simulink model "Grid_ModelSimVSGConB"  (R2025b)
settings: Solver=daessc  StartTime=0.0  StopTime=10  MaxStep=1e-5  RelTol=1e-3
InitFcn:
  | Grid_ModelSimV1
values from neighbouring files (symbols this model uses):
  a = 0.5    [Grid_ModelSimV1.m]
  b = (beta*gamma)/(beta + gamma - a)    [Grid_ModelSimV1.m]
  c = (beta + gamma - a)/mp    [Grid_ModelSimV1.m]
  D1 = Moh_Dp/Moh_Sbase    (= 0.2546)    [Grid_ModelSimV1.m]
  D2 = 0.4    [Grid_ModelSimV1.m]
  delta1_0 = delta1PCC0 + atan2(      P12_0*X1/V1PCCmag0,      V1PCCmag0 + Q12_0*X1/V1PCCmag0 )    [Grid_ModelSimV1.m]
  delta2_0 = delta2PCC0 + atan2(      Pm2_0*X2/V2PCCmag0,      V2PCCmag0 + Q21_0*X2/V2PCCmag0 )    [Grid_ModelSimV1.m]
  Dw1_0 = 0    [Grid_ModelSimV1.m]
  Dw2_0 = 0    [Grid_ModelSimV1.m]
  E2_0 = hypot(      Pm2_0*X2/V2PCCmag0,      V2PCCmag0 + Q21_0*X2/V2PCCmag0 )    [Grid_ModelSimV1.m]
  H1 = J*omega_nom^2/2    (= 39.9916370332)    [Grid_ModelSimV1.m]
  H2 = 12    [Grid_ModelSimV1.m]
  Imax = 1.20    (= 1.2)    [Grid_ModelSimV1.m]
  J = Moh_J/Moh_Sbase    (= 0.0008104)    [Grid_ModelSimV1.m]
  Ki = 0.5    [Grid_ModelSimV1.m]
  Kiq = Moh_Kiq*Moh_Sbase/Moh_Vbase    [Grid_ModelSimV1.m]
  Lf = 1e-3    (= 0.001)    [Grid_ModelSimV1.m]
  LimitEnable = 1    [Grid_ModelSimV1.m]
  Ls = Xs/ws    [Grid_ModelSimV1.m]
  Ls_line = Xs_line/ws    [Grid_ModelSimV1.m]
  nq = Moh_nq*Moh_Sbase/Moh_Vbase    [Grid_ModelSimV1.m]
  omega_nom = ws    (= 314.159265359)    [Grid_ModelSimV1.m]
  Pload_0 = P12_0    (= 1)    [Grid_ModelSimV1.m]
  Qref = 0.0    (= 0)    [Grid_ModelSimV1.m]
  Rf = 1.0    (= 1)    [Grid_ModelSimV1.m]
  RLFault = 0    [Grid_ModelSimV1.m]
  Rs = Zs_mag/sqrt(1 + XR_grid^2)    [Grid_ModelSimV1.m]
  Rs_line = GridLineFraction*Rs    [Grid_ModelSimV1.m]
  SolidFault = 0    [Grid_ModelSimV1.m]
  ws = 2*pi*f    (= 314.159265359)    [Grid_ModelSimV1.m]
  X1 = Xtf_src_total_pu    (= 0.15)    [Grid_ModelSimV1.m]
libraries: nesl_utility x87, ee_lib x78, fl_lib x40, eePowerMeasurement x7
(part 3 of 6)

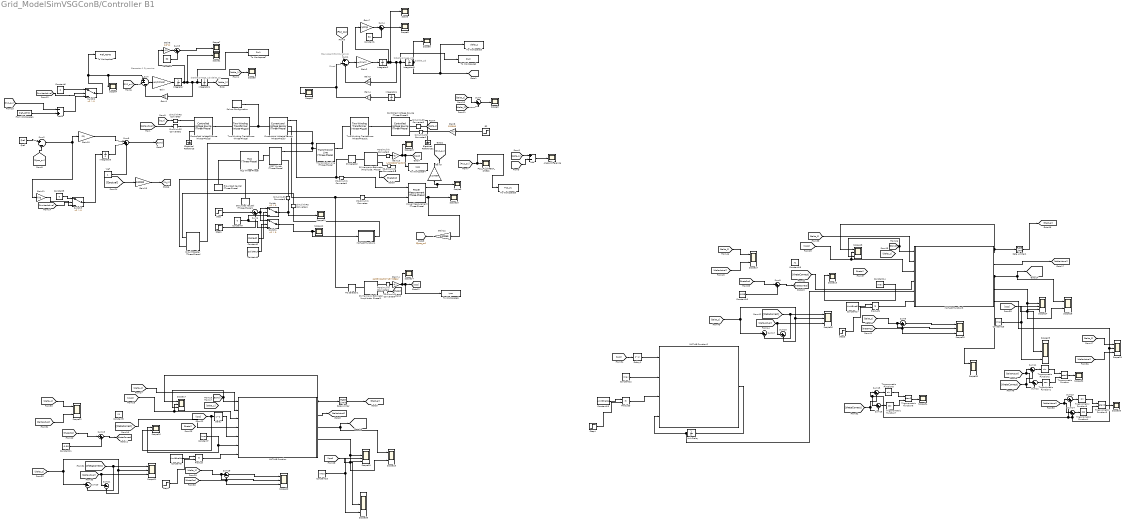
== system Grid_ModelSimVSGConB/Controller B1 ==
  note: Pload
  note: Equivalent Grid Dynamics
  note: $\delta_1$
  note: $\Delta\omega_1$
  note: Generator 1 Dynamics
  note: $\Delta\omega_2$
  note: $\delta_2$
  Add : Sum  Inputs=+-
  Add3 : Sum  Inputs=-+
  Angle Difference : Scope
      settings: ActiveDisplayYMinimum=-1797.079300536021  ActiveDisplayYMaximum=1392.8706624711849  DataLoggingVariableName=ScopeData11
  Circuit Breaker (Three-Phase) : ee_lib/Switches & Breakers/Circuit Breaker (Three-Phase)  R_closed=0.001 Ohm  G_open=1e-6 1/Ohm  threshold=0.5 V  breaker_behavior=ee.enum.switches.breakerBehavior.zeroCrossingEnable
      settings: InternalSimscapePortConfiguration="{\"Bottom\":[],\"Left\":[{\"id\":\"vT\",\"label\":\"vT\",\"type\":\"input\"},{\"id\":\"N1\",\"label\":\"~1\",\"type\":\"foundation.electrical.three_phase\"}],\"Right\":[{\"id\":\"N2\",\"label\":\"~2\",\"type\":\"foundation.electrical.three_phase\"}],\"Top\":[]}"
  Constant : Constant  Value=50
  Constant1 : Constant  Value=50
  Constant{7,10,12,14..15} (5 alike) : Constant  Value=Imax
  Constant11 : Constant  Value=-0.58
  Constant13 : Constant  Value=LimitEnable
  Constant16 : Constant  Value=-0.58
  Constant17 : Constant  Value=LimitEnable
  Constant18 : Constant  Value=X1
  Constant2 : Constant  Value=RLFault
  Constant3 : Constant  Value=SolidFault
  Constant4 : Constant  Value=0
  Constant5 : Constant  Value=0
  Constant6 : Constant  Value=0
  Constant8 : Constant  Value=LimitEnable
  Constant9 : Constant  Value=X1
  Controlled Voltage Source (Three-Phase) : ee_lib/Sources/Controlled Voltage Source (Three-Phase)  input_option=ee.enum.inputType.singleFreqAC  FRated=50 Hz
      settings: InternalSimscapePortConfiguration="{\"Bottom\":[],\"Left\":[{\"id\":\"Vt\",\"label\":\"Vt\",\"type\":\"input\"},{\"id\":\"ph\",\"label\":\"ph\",\"type\":\"input\"},{\"id\":\"n\",\"label\":\"n\",\"type\":\"foundation.electrical.electrical\"}],\"Right\":[{\"id\":\"N\",\"label\":\"~\",\"type\":\"foundation.electrical.three_phase\"}],\"Top\":[]}"
  Controlled Voltage Source (Three-Phase)1 : ee_lib/Sources/Controlled Voltage Source (Three-Phase)  input_option=ee.enum.inputType.singleFreqAC  FRated=50 Hz
      settings: InternalSimscapePortConfiguration="{\"Bottom\":[],\"Left\":[{\"id\":\"Vt\",\"label\":\"Vt\",\"type\":\"input\"},{\"id\":\"ph\",\"label\":\"ph\",\"type\":\"input\"},{\"id\":\"n\",\"label\":\"n\",\"type\":\"foundation.electrical.electrical\"}],\"Right\":[{\"id\":\"N\",\"label\":\"~\",\"type\":\"foundation.electrical.three_phase\"}],\"Top\":[]}"
  Current and Voltage Sensor (Three-Phase) : ee_lib/Sensors & Transducers/Current and Voltage Sensor (Three-Phase)  vMeasurementType=ee.enum.vmeasurement.ll  outputUnit=ee.enum.unit.si  SRated=100e6 A*V  VRated=24e3 V  I_specify=off  I_priority=None  I=[0, 0, 0] A  I_nominal_specify=off  I_nominal_value=1  I_nominal_unit=A  V_specify=off  V_priority=None  V=[0, 0, 0] V  V_nominal_specify=off  V_nominal_value=1  V_nominal_unit=V
      settings: InternalSimscapePortConfiguration="{\"Bottom\":[],\"Left\":[{\"id\":\"N1\",\"label\":\"~1\",\"type\":\"foundation.electrical.three_phase\"}],\"Right\":[{\"id\":\"V_output\",\"label\":\"V\",\"type\":\"output\"},{\"id\":\"I_output\",\"label\":\"I\",\"type\":\"output\"},{\"id\":\"N2\",\"label\":\"~2\",\"type\":\"foundation.electrical.three_phase\"}],\"Top\":[]}"
  Delay : Delay  InitialCondition=1  SampleTime=1e-4
  Delay1 : Delay  InitialCondition=1  SampleTime=1e-4
  E2 : Step  Before=E2_0  After=E2_0  SampleTime=0
  Electrical Reference : fl_lib/Electrical/Electrical Elements/Electrical Reference
  Electrical Reference1 : fl_lib/Electrical/Electrical Elements/Electrical Reference
  From Workspace1 : FromWorkspace  VariableName=Pref_AEMO  Interpolate=off  OutputAfterFinalValue=Holding final value
  Gain : Gain  Gain=ws/(2*H1)
  Gain1 : Gain  Gain=D1
  Gain10 : Gain  Gain=nq
  Gain11 : Gain  Gain=Kiq
  Gain12 : Gain  Gain=1/100e6
  Gain13 : Gain  Gain=1/(132000*sqrt(2))
  Gain14 : Gain  Gain=sqrt(3)/(sqrt(2)*437.3866)
  Gain15 : Gain  Gain=132000
  Gain2 : Gain  Gain=ws/(2*H2)
  Gain3 : Gain  Gain=D2
  Gain4 : Gain  Gain=Ki
  Gain5 : Gain  Gain=1/100e6
  Gain6 : Gain  Gain=1/2*pi
  Gain7 : Gain  Gain=1/2*pi
  Gain8 : Gain  Gain=132000
  Grounded Neutral (Three-Phase) : ee_lib/Connectors & References/Grounded Neutral (Three-Phase)
  Grounded Neutral (Three-Phase)1 : ee_lib/Connectors & References/Grounded Neutral (Three-Phase)
  Integrator : Integrator  InitialCondition=Dw1_0
  Integrator1 : Integrator  InitialCondition=delta1_0
  Integrator2 : Integrator  InitialCondition=Dw2_0
  Integrator3 : Integrator  InitialCondition=delta2_0
  Integrator4 : Integrator  InitialCondition=Pload_0/Ki
  Integrator5 : Integrator
  MATLAB Function : MATLAB Function  TreatAsAtomicUnit=on
  MATLAB Function1 : MATLAB Function  TreatAsAtomicUnit=on
  MATLAB Function2 : MATLAB Function  TreatAsAtomicUnit=on
  MATLAB Function3 : MATLAB Function  TreatAsAtomicUnit=on
  P12_PU_DIRECT_CHECK : Scope
      settings: ActiveDisplayYMinimum=0.025769954116994787  ActiveDisplayYMaximum=1.1382760295145928  DataLoggingVariableName=ScopeData3
  "PS Harmonic Estimator (Amplitude, Phase)" : fl_lib/Physical Signals/Periodic Operators/PS Harmonic Estimator (Amplitude, Phase)  f0=50 Hz  n=1  amplMin=0.001 V
      settings: InternalSimscapePortConfiguration="{\"Bottom\":[],\"Left\":[{\"id\":\"I\",\"label\":\"I\",\"type\":\"input\"}],\"Right\":[{\"id\":\"A\",\"label\":\"A\",\"type\":\"output\"},{\"id\":\"Phi\",\"label\":\"Phi\",\"type\":\"output\"}],\"Top\":[]}"
  "PS Harmonic Estimator (Amplitude, Phase)1" : fl_lib/Physical Signals/Periodic Operators/PS Harmonic Estimator (Amplitude, Phase)  f0=50 Hz  n=1  amplMin=0.001 A
      settings: InternalSimscapePortConfiguration="{\"Bottom\":[],\"Left\":[{\"id\":\"I\",\"label\":\"I\",\"type\":\"input\"}],\"Right\":[{\"id\":\"A\",\"label\":\"A\",\"type\":\"output\"},{\"id\":\"Phi\",\"label\":\"Phi\",\"type\":\"output\"}],\"Top\":[]}"
  PS Selector : fl_lib/Physical Signals/Nonlinear Operators/PS Selector  ix=1
      settings: InternalSimscapePortConfiguration="{\"Bottom\":[],\"Left\":[{\"id\":\"I\",\"label\":\"\",\"type\":\"input\"}],\"Right\":[{\"id\":\"O\",\"label\":\"\",\"type\":\"output\"}],\"Top\":[]}"
  PS Selector1 : fl_lib/Physical Signals/Nonlinear Operators/PS Selector  ix=1
      settings: InternalSimscapePortConfiguration="{\"Bottom\":[],\"Left\":[{\"id\":\"I\",\"label\":\"\",\"type\":\"input\"}],\"Right\":[{\"id\":\"O\",\"label\":\"\",\"type\":\"output\"}],\"Top\":[]}"
  PS-Simulink Converter{,1..5} (6 alike) : nesl_utility/PS-Simulink Converter  PhysicalDomain=network_engine_domain  SubClassName=ps_output  LeftPortType=input  RightPortType=output  PseudoPeriodic=off  Frequencies=[]  VectorFormat=inherit  Unit=inherit  AffineConversion=off
  Power Measurement (Three-Phase) : eePowerMeasurement/Power Measurement (Three-Phase)  LabelModeActiveChoice=Continuous  F=50  K=1  Seq=Positive  Ts=0
  Product : Product
  Product1 : Product
  Product3 : Product
  Qref : Constant  Value=Qref
  RLC (Three-Phase) : ee_lib/Passive/RLC Assemblies/RLC (Three-Phase)  port_option=ee.enum.threePhasePort.composite  component_structure=ee.enum.rlc.structure.SeriesRL  R=Rf Ohm  L=Lf H  C=1e-6 F  R_parasitic=0 Ohm  G_parasitic=0 1/Ohm  IL_specify=off  IL_priority=High  IL=[0, 0, 0] A  IL_nominal_specify=off  IL_nominal_value=1  IL_nominal_unit=A  VC_specify=off  VC_priority=High  VC=[0, 0, 0] V  VC_nominal_specify=off  VC_nominal_value=1  VC_nominal_unit=V
      settings: InternalSimscapePortConfiguration="{\"Bottom\":[],\"Left\":[{\"id\":\"N1\",\"label\":\"~1\",\"type\":\"foundation.electrical.three_phase\"}],\"Right\":[{\"id\":\"N2\",\"label\":\"~2\",\"type\":\"foundation.electrical.three_phase\"}],\"Top\":[]}"
  Rate Limiter : RateLimiter  RisingSlewLimit=5  FallingSlewLimit=-1000  SampleTimeMode=inherited
  Rate Limiter1 : RateLimiter  RisingSlewLimit=5  FallingSlewLimit=-1000  SampleTimeMode=inherited
  SPST Switch (Three-Phase) : ee_lib/Switches & Breakers/SPST Switch (Three-Phase)  R_closed=0.001 Ohm  G_open=1e-6 1/Ohm  threshold=0.5 V  i_vT_specify=off  i_vT_priority=None  i_vT=0 A  i_vT_nominal_specify=off  i_vT_nominal_value=1  i_vT_nominal_unit=A  I_specify=off  I_priority=None  I=[0, 0, 0] A  I_nominal_specify=off  I_nominal_value=1  I_nominal_unit=A  V_specify=off  V_priority=None  V=[0, 0, 0] V  V_nominal_specify=off  V_nominal_value=1  V_nominal_unit=V  i_a_specify=off  i_a_priority=None  i_a=0 A  i_a_nominal_specify=off  i_a_nominal_value=1  i_a_nominal_unit=A  v_a_specify=off  v_a_priority=None  v_a=0 V  v_a_nominal_specify=off  v_a_nominal_value=1  v_a_nominal_unit=V  i_b_specify=off  i_b_priority=None  i_b=0 A  i_b_nominal_specify=off  i_b_nominal_value=1  i_b_nominal_unit=A  v_b_specify=off  v_b_priority=None  v_b=0 V  v_b_nominal_specify=off  v_b_nominal_value=1  v_b_nominal_unit=V  i_c_specify=off  i_c_priority=None  i_c=0 A  i_c_nominal_specify=off  i_c_nominal_value=1  i_c_nominal_unit=A  v_c_specify=off  v_c_priority=None  v_c=0 V  v_c_nominal_specify=off  v_c_nominal_value=1  v_c_nominal_unit=V
      settings: InternalSimscapePortConfiguration="{\"Bottom\":[],\"Left\":[{\"id\":\"vT\",\"label\":\"vT\",\"type\":\"input\"},{\"id\":\"N1\",\"label\":\"~1\",\"type\":\"foundation.electrical.three_phase\"}],\"Right\":[{\"id\":\"N2\",\"label\":\"~2\",\"type\":\"foundation.electrical.three_phase\"}],\"Top\":[]}"
  Scope{,1..14,32..34} (18 alike) : Scope
      Scope10 settings: ActiveDisplayYMinimum=-7.0875379074731711E+6  ActiveDisplayYMaximum=3.5866343126415364E+7  DataLoggingVariableName=ScopeData10
      Scope11 settings: ActiveDisplayYMinimum=-1  ActiveDisplayYMaximum=1  DataLoggingVariableName=ScopeData12
      Scope12 settings: ActiveDisplayYMinimum=-0.099895670318205565  ActiveDisplayYMaximum=1.090580520157985  DataLoggingVariableName=ScopeData13
      Scope13 settings: ActiveDisplayYMinimum=-2.5658886223026931  ActiveDisplayYMaximum=3.94553749363296  DataLoggingVariableName=ScopeData17
      Scope14 settings: ActiveDisplayYMinimum=-1.0313612715858387  ActiveDisplayYMaximum=9.28225144427255  DataLoggingVariableName=ScopeData49
      Scope2 settings: ActiveDisplayYMinimum=-1.1623447136135812  ActiveDisplayYMaximum=1.3781315704633705  DataLoggingVariableName=ScopeData2
      Scope3 settings: ActiveDisplayYMinimum=-6.9165953549105517  ActiveDisplayYMaximum=7.2970312476918844  DataLoggingVariableName=ScopeData23
      Scope32 settings: ActiveDisplayYMinimum=-3.9269892876580919  ActiveDisplayYMaximum=3.9269891159141448  DataLoggingVariableName=ScopeData60
      Scope33 settings: ActiveDisplayYMinimum=-1  ActiveDisplayYMaximum=1  DataLoggingVariableName=ScopeData61
      Scope34 settings: ActiveDisplayYMinimum=-1.4401977699145856  ActiveDisplayYMaximum=2.6200072427590877  DataLoggingVariableName=ScopeData62
      Scope4 settings: ActiveDisplayYMinimum=-0.10712539123630682  ActiveDisplayYMaximum=1.1397496087636934  DataLoggingVariableName=ScopeData4
      Scope5 settings: ActiveDisplayYMinimum=-0.5315157226665419  ActiveDisplayYMaximum=2.1795261958257051  DataLoggingVariableName=ScopeData5
      Scope6 settings: DataLoggingVariableName=ScopeData6
      Scope7 settings: ActiveDisplayYMinimum=49.687624753361064  ActiveDisplayYMaximum=50.693198364995283  DataLoggingVariableName=ScopeData7
      Scope8 settings: ActiveDisplayYMinimum=49.92788610274394  ActiveDisplayYMaximum=50.170097472488152  DataLoggingVariableName=ScopeData8
      Scope9 settings: ActiveDisplayYMinimum=-1.0746752531857479E+8  ActiveDisplayYMaximum=3.4916793473002666E+8  DataLoggingVariableName=ScopeData9
  Scope{15..16,22..23,27..28,30} (7 alike) : Scope  NumInputPorts=2
      Scope15 settings: ActiveDisplayYMinimum=-1.1863011737345548  ActiveDisplayYMaximum=10.676710563610996  DataLoggingVariableName=ScopeData50
      Scope16 settings: ActiveDisplayYMinimum=-1.1863011737345548  ActiveDisplayYMaximum=10.676710563610996  DataLoggingVariableName=ScopeData63
      Scope22 settings: ActiveDisplayYMinimum=-0.789059573220128  ActiveDisplayYMaximum=0.68498191992001933  DataLoggingVariableName=ScopeData68
      Scope23 settings: ActiveDisplayYMinimum=-0.12499999999999997  ActiveDisplayYMaximum=1.125  DataLoggingVariableName=ScopeData69
      Scope27 settings: ActiveDisplayYMinimum=-3.7225747393161841  ActiveDisplayYMaximum=4.13168438536474  DataLoggingVariableName=ScopeData55
      Scope28 settings: ActiveDisplayYMinimum=-0.12499999999999997  ActiveDisplayYMaximum=1.125  DataLoggingVariableName=ScopeData56
      Scope30 settings: ActiveDisplayYMinimum=-0.12499999999999997  ActiveDisplayYMaximum=1.125  DataLoggingVariableName=ScopeData58
  Scope{17..18,20..21,25..26,29,31,35} (9 alike) : Scope  NumInputPorts=3
      Scope17 settings: ActiveDisplayYMinimum=-0.15152887647529475  ActiveDisplayYMaximum=1.3637598882776532  DataLoggingVariableName=ScopeData64
      Scope18 settings: ActiveDisplayYMinimum=-0.12862546618818504  ActiveDisplayYMaximum=1.1576291956936657  DataLoggingVariableName=ScopeData51
      Scope20 settings: ActiveDisplayYMinimum=-2.6035343832796971  ActiveDisplayYMaximum=9.8526279409331341  DataLoggingVariableName=ScopeData66
      Scope21 settings: ActiveDisplayYMinimum=-2.7720251649113785  ActiveDisplayYMaximum=1.647845241487004  DataLoggingVariableName=ScopeData67
      Scope25 settings: ActiveDisplayYMinimum=-2.6035343832796971  ActiveDisplayYMaximum=9.8526279409331341  DataLoggingVariableName=ScopeData53
      Scope26 settings: ActiveDisplayYMinimum=-2.7720251649113785  ActiveDisplayYMaximum=1.647845241487004  DataLoggingVariableName=ScopeData54
      Scope29 settings: ActiveDisplayYMinimum=-0.5707391589619073  ActiveDisplayYMaximum=5.1366524306571666  DataLoggingVariableName=ScopeData57
      Scope31 settings: ActiveDisplayYMinimum=-2.7504004579249388  ActiveDisplayYMaximum=0.52931298913436242  DataLoggingVariableName=ScopeData59
      Scope35 settings: ActiveDisplayYMinimum=-1.0836921534712509  ActiveDisplayYMaximum=9.974041191278685  DataLoggingVariableName=ScopeData70
  Scope19 : Scope  NumInputPorts=4
      settings: ActiveDisplayYMinimum=-0.9517189141745912  ActiveDisplayYMaximum=8.9949029547267862  DataLoggingVariableName=ScopeData65
  Scope24 : Scope  NumInputPorts=4
      settings: ActiveDisplayYMinimum=-0.17065097766172704  ActiveDisplayYMaximum=1.5358587989555437  DataLoggingVariableName=ScopeData52
  Simulink-PS Converter{,1..5} (6 alike) : nesl_utility/Simulink-PS Converter  PhysicalDomain=network_engine_domain  SubClassName=ps_input  LeftPortType=input  RightPortType=output  PseudoPeriodic=off  Frequencies=[]  NoiseDistribution=none  NoiseParameters=[]  Unit=1  AffineConversion=off  FilteringAndDerivatives=provide  SimscapeFilterOrder=1  InputFilterTimeConstant=0.001  UdotUserProvided=0
  Solver Configuration : nesl_utility/Solver Configuration  PhysicalDomain=network_engine_domain  SubClassName=solver  LeftPortType=input  RightPortType=generic  Tones=[]  Harmonics=[]  SimulateNoise=off  Profile=off  UseLocalSampling=off  EnableSwitchedLinearOptims=on  FrequencyDomain=off  UseCCode=off  RelTol=0.001  AbsTol=0.001  MinStep=1e-09  ToWorkspace=off  RevertToSquareIcSolve=off  NumHomotopyIterations=100  PhasorMode=off  PhasorModeNumHarmonics=1  ConsistencySolver=NEWTON_XTOL_AFTER_FTOL  IndexReductionMethod=DerivativeReplacement  DoDC=off  ResidualTolerance=1e-09  ConsistencyTolSource=GLOBAL  ConsistencyAbsTol=0.001  ConsistencyRelTol=0.001  ConsistencyTolFactor=0.001  UseLocalSolver=off  LocalSolverChoice=NE_BACKWARD_EULER_ADVANCER  ResolveIndetEquations=on  FunctionEvalNumThread=1  LocalSolverSampleTime=0.001  DoFixedCost=off  MaxNonlinIter=3  MaxModeIter=2  ComputeImpulses=off  ImpulseIterations=2  LinearAlgebra=auto  LinearAlgebraNumThread=0  EquationFormulation=NE_TIME_EF  DelaysMemoryBudget=1024  AutomaticFiltering=on  FilteringTimeConstant=0.001  PartitionStorageMethod=AS_NEEDED  PartitionMemoryBudget=1024  PartitionMethod=ROBUST  MultibodyUseLocalSolver=off  MultibodyLocalSolverChoice=ODE1  MultibodyLocalSolverSampleTime=0.001
  Step : Step  Time=5  SampleTime=0
  Step1 : Step  Time=5.43  After=-1  SampleTime=0
  Step2 : Step  Time=3  SampleTime=0
  Step3 : Step  Time=3  SampleTime=0
  Step4 : Step  Time=3  SampleTime=0
  Sum : Sum  Inputs=|+|-|-
  Sum1 : Sum  Inputs=|+|-|-
  Sum{7..8,10..18,20..21} (13 alike) : Sum  Inputs=|+-
  Sum{3..4,6,9,19} (5 alike) : Sum  Inputs=|++
  Sum2 : Sum  Inputs=|+|-
  Sum5 : Sum  Inputs=|+++
  Switch{,1..3} (4 alike) : Switch  Criteria=u2 > Threshold  SaturateOnIntegerOverflow=off  InputSameDT=off
  To Workspace1 : ToWorkspace  VariableName=Pref_AEMO  SaveFormat=Timeseries  SampleTime=-1
  To Workspace2 : ToWorkspace  VariableName=Dw2  SaveFormat=Timeseries  SampleTime=-1
  To Workspace3 : ToWorkspace  VariableName=delta_2  SaveFormat=Timeseries  SampleTime=-1
  To Workspace4 : ToWorkspace  VariableName=Vpcc  SaveFormat=Timeseries  SampleTime=-1
  To Workspace5 : ToWorkspace  VariableName=P12_pu  SaveFormat=Timeseries  SampleTime=-1
  To Workspace6 : ToWorkspace  VariableName=Ipcc  SaveFormat=Timeseries  SampleTime=-1
  To Workspace7 : ToWorkspace  VariableName=Dw1  SaveFormat=Timeseries  SampleTime=-1
  Transmission Line (Three-Phase) : ee_lib/Passive/Lines/Transmission Line (Three-Phase)  length=1 km  freq=f Hz  R=Rs_line Ohm/km  L=Ls_line*1000 mH/km  M=0 mH/km  Cl=0.3 uF/km  Cg=0.1 uF/km  Rm=0 Ohm/km  ModelTwoSections=ee.enum.enable.no  N=1  InterfacePosition=0.5 km  N1sec=1  N2sec=1  Access_ground=ee.enum.enable.no  R_parasitic=1e-6 Ohm  G_parasitic=1e-6 1/Ohm
      settings: InternalSimscapePortConfiguration="{\"Bottom\":[],\"Left\":[{\"id\":\"N1\",\"label\":\"~1\",\"type\":\"foundation.electrical.three_phase\"},{\"id\":\"g1\",\"label\":\"g1\",\"type\":\"foundation.electrical.electrical\"}],\"Right\":[{\"id\":\"N2\",\"label\":\"~2\",\"type\":\"foundation.electrical.three_phase\"},{\"id\":\"g2\",\"label\":\"g2\",\"type\":\"foundation.electrical.electrical\"}],\"Top\":[]}"
  Trigonometric Function : Trigonometry  Operator=atan2
  Trigonometric Function1 : Trigonometry  Operator=cos
  Trigonometric Function2 : Trigonometry
  Trigonometric Function3 : Trigonometry  Operator=atan2
  Trigonometric Function4 : Trigonometry  Operator=cos
  Trigonometric Function5 : Trigonometry
  Trigonometric Function6 : Trigonometry  Operator=atan2
  Trigonometric Function7 : Trigonometry  Operator=cos
  Trigonometric Function8 : Trigonometry
  Two-Winding Transformer (Three-Phase) : ee_lib/Passive/Transformers/Two-Winding Transformer (Three-Phase)  SRated=100e6 A*V  FRated=50 Hz  Winding1Connection=ee.enum.windingconnection.Yg  VRated1=132000 V  Winding2Connection=ee.enum.windingconnection.Yg  VRated2=132000 V  CoreType=ee.enum.coretype.threelimb  pu_Rw1=Rtf_src_pri_pu  pu_Rw2=Rtf_src_sec_pu  leakage_reactance_option=ee.enum.transformer_leakage.include  pu_Xl1=Xtf_src_pri_pu  pu_Xl2=Xtf_src_sec_pu  magnetizing_resistance_option=ee.enum.transformer_magnetizingResistance.exclude  pu_Rm=500  magnetizing_reactance_option=ee.enum.transformer_magnetizingReactance.exclude  saturation_option=ee.enum.transformer_saturation.exclude  pu_Xm=500  current_data=[0, .002, 1, 2]  magnetic_flux_data=[0, 1.2, 1.5, 1.51]  pu_X0=0.5  i1_specify=off  i1_priority=None  i1=[0, 0, 0] A  i1_nominal_specify=off  i1_nominal_value=1  i1_nominal_unit=A  i2_specify=off  i2_priority=None  i2=[0, 0, 0] A  i2_nominal_specify=off  i2_nominal_value=1  i2_nominal_unit=A  phi_specify=off  phi_priority=None  phi=[0, 0, 0]  phi_nominal_specify=off  phi_nominal_value=1  phi_nominal_unit=1  power_dissipated_specify=off  power_dissipated_priority=None  power_dissipated=0 W  power_dissipated_nominal_specify=off  power_dissipated_nominal_value=1  power_dissipated_nominal_unit=W
      settings: InternalSimscapePortConfiguration="{\"Bottom\":[],\"Left\":[{\"id\":\"N1\",\"label\":\"~1\",\"type\":\"foundation.electrical.three_phase\"}],\"Right\":[{\"id\":\"N2\",\"label\":\"~2\",\"type\":\"foundation.electrical.three_phase\"}],\"Top\":[]}"
  Two-Winding Transformer (Three-Phase)1 : ee_lib/Passive/Transformers/Two-Winding Transformer (Three-Phase)  SRated=100e6 A*V  FRated=50 Hz  Winding1Connection=ee.enum.windingconnection.Y  VRated1=132000 V  Winding2Connection=ee.enum.windingconnection.Y  VRated2=132000 V  CoreType=ee.enum.coretype.threelimb  pu_Rw1=Rtf_grid_pri_pu  pu_Rw2=Rtf_grid_sec_pu  leakage_reactance_option=ee.enum.transformer_leakage.include  pu_Xl1=Xtf_grid_pri_pu  pu_Xl2=Xtf_grid_sec_pu  magnetizing_resistance_option=ee.enum.transformer_magnetizingResistance.exclude  pu_Rm=500  magnetizing_reactance_option=ee.enum.transformer_magnetizingReactance.exclude  saturation_option=ee.enum.transformer_saturation.exclude  pu_Xm=500  current_data=[0, .002, 1, 2]  magnetic_flux_data=[0, 1.2, 1.5, 1.51]  pu_X0=0.5  i1_specify=off  i1_priority=None  i1=[0, 0, 0] A  i1_nominal_specify=off  i1_nominal_value=1  i1_nominal_unit=A  i2_specify=off  i2_priority=None  i2=[0, 0, 0] A  i2_nominal_specify=off  i2_nominal_value=1  i2_nominal_unit=A  phi_specify=off  phi_priority=None  phi=[0, 0, 0]  phi_nominal_specify=off  phi_nominal_value=1  phi_nominal_unit=1  power_dissipated_specify=off  power_dissipated_priority=None  power_dissipated=0 W  power_dissipated_nominal_specify=off  power_dissipated_nominal_value=1  power_dissipated_nominal_unit=W
      settings: InternalSimscapePortConfiguration="{\"Bottom\":[],\"Left\":[{\"id\":\"N1\",\"label\":\"~1\",\"type\":\"foundation.electrical.three_phase\"}],\"Right\":[{\"id\":\"N2\",\"label\":\"~2\",\"type\":\"foundation.electrical.three_phase\"}],\"Top\":[]}"
  Unit Delay : UnitDelay  InitialCondition=1  SampleTime=1e-4  HasFrameUpgradeWarning=on
  Vref : Constant
  wires:
  Switch/1 -> Simulink-PS Converter5/1, Scope11/1
  Step1/1 -> Sum6/2
  Constant4/1 -> Switch1/3, Switch/3
  [P12_pu] -> To Workspace5/1, P12_PU_DIRECT_CHECK/1
  Power Measurement (Three-Phase)/2 -> Scope10/1, Gain12/1
  Gain3/1 -> Sum1/3
  Gain5/1 -> [P12_pu]
  Sum/1 -> Gain/1
  [Qpcc_pu] -> Sum2/2
  Sum6/1 -> Switch1/1, Switch/1
  Add/1 -> Angle Difference/1
  PS-Simulink Converter1/1 -> Power Measurement (Three-Phase)/1
  Constant3/1 -> Switch1/2
  Gain8/1 -> Simulink-PS Converter1/1
  Sum1/1 -> Gain2/1
  Integrator5/1 -> Sum5/2
  Qref/1 -> Sum2/1
  [delta_2] -> Add/2
  Gain1/1 -> Sum/3
  E2/1 -> Gain8/1
  Gain6/1 -> Sum3/1
  Integrator2/1 -> Gain7/1, Scope/1, Gain3/1, To Workspace2/1, Integrator3/1, Integrator4/1
  [Vt_V] -> Simulink-PS Converter/1
  Gain/1 -> Integrator/1
  PS-Simulink Converter/1 -> Power Measurement (Three-Phase)/2
  Integrator4/1 -> Gain4/1
  Constant/1 -> Sum3/2
  Gain4/1 -> Scope2/1, Sum1/2
  Constant1/1 -> Sum4/2
  [deltaActual] -> Simulink-PS Converter2/1
  [P12_pu] -> Sum/2
  Gain12/1 -> [Qpcc_pu]
  Sum5/1 -> [Ecmd]
  Gain2/1 -> Integrator2/1
  Sum2/1 -> Gain11/1, Gain10/1
  [delta_2] -> Simulink-PS Converter3/1
  Vref/1 -> Sum5/3
  Gain10/1 -> Sum5/1
  [delta_1] -> Scope5/1
  Sum4/1 -> Scope8/1
  Integrator1/1 -> [delta_1]
  Switch3/1 -> Integrator5/1
  Gain7/1 -> Sum4/1
  Switch2/1 -> To Workspace1/1, Sum/1, Scope4/1
  Power Measurement (Three-Phase)/1 -> Scope9/1, Gain5/1  "P12 (SimEl)"
  Sum3/1 -> Scope7/1
  [delta_1] -> Add/1
  [P12_pu] -> Sum1/1
  Step/1 -> Sum6/1
  Switch1/1 -> MATLAB Function1/1(u), Scope12/1
  Constant2/1 -> Switch/2
  PS-Simulink Converter2/1 -> Gain13/1
  Gain13/1 -> Scope13/1, To Workspace4/1, [Vpcc]
  Integrator/1 -> Gain6/1, Scope1/1, To Workspace7/1, Integrator1/1, Gain1/1
  Integrator3/1 -> [delta_2], To Workspace3/1, Scope6/1
  [delta_1] -> Sum7/1
  [delta_2] -> Sum7/2
  Sum7/1 -> Scope3/1
  PS-Simulink Converter5/1 -> [thetaI]
  PS-Simulink Converter4/1 -> Gain14/1
  Gain14/1 -> To Workspace6/1, [Ipcc], Scope14/1
  Add3/1 -> Switch2/3
  [P12_pu] -> Add3/1
  Constant6/1 -> Switch2/1
  [LimiterActive] -> Switch2/2
  From Workspace1/1 -> Add3/2
  [LimiterActive] -> Switch3/2
  Constant5/1 -> Switch3/1
  Gain11/1 -> Switch3/3
  PS-Simulink Converter3/1 -> [thetaPcc]
  [Eactual] -> Gain15/1
  MATLAB Function1/1(y) -> Simulink-PS Converter4/1
  [thetaPcc] -> Sum9/1
  MATLAB Function3/2(deltaActual) -> [deltaActual]
  Trigonometric Function7/1 -> Trigonometric Function6/2
  Trigonometric Function6/1 -> Scope34/1
  [delta_1] -> Scope31/1
  [delta_1] -> MATLAB Function3/2(deltaCmd)
  Step3/1 -> Product1/2
  Step4/1 -> Product3/2
  [thetaCorrect] -> MATLAB Function3/4(deltaPCC)
  Constant15/1 -> Scope29/3, Scope24/3
  MATLAB Function3/5(deltaPCC_used) -> Sum13/2, Sum15/1, Sum16/1, Sum14/2, Scope31/2
  [Ipcc] -> Delay1/1
  Sum15/1 -> Trigonometric Function8/1
  Constant13/1 -> Product3/1
  [deltaActual] -> Scope31/3
  Trigonometric Function/1 -> Scope32/1
  [deltaActual] -> Sum10/1, Scope26/3
  Sum9/1 -> [thetaCorrect]
  Trigonometric Function3/1 -> Scope33/1
  [thetaCorrect] -> Sum12/2, Sum11/2
  Sum12/1 -> Trigonometric Function1/1
  [delta_1] -> Scope27/1
  Rate Limiter1/1 -> [Eactual]
  Constant14/1 -> Scope15/1
  [Vpcc] -> Scope18/2, MATLAB Function3/3(Vpcc)
  [Ecmd] -> Scope18/3, MATLAB Function3/1(Ecmd)
  Delay1/1 -> MATLAB Function2/1(Imeas)
  Constant16/1 -> Sum9/2
  Sum14/1 -> Trigonometric Function4/1
  Trigonometric Function2/1 -> Trigonometric Function/1
  MATLAB Function3/4(scale) -> Scope28/2, Scope24/2
  Constant12/1 -> MATLAB Function2/2(Imax)
  Trigonometric Function8/1 -> Trigonometric Function6/1
  [Ipcc] -> Scope29/2, Scope24/4
  [deltaActual] -> Sum12/1, Sum11/1
  Unit Delay/1 -> MATLAB Function3/5(kApplied), MATLAB Function2/4(kPrev)
  Product3/1 -> MATLAB Function2/3(LimitEnable)
  [deltaActual] -> Sum14/1, Sum13/1
  MATLAB Function3/3(LimiterActive) -> Scope30/1, [LimiterActive], Scope28/1
  Sum11/1 -> Trigonometric Function2/1
  [delta_1] -> Sum17/1, Sum10/2, Scope26/2
  Trigonometric Function5/1 -> Trigonometric Function3/1
  Trigonometric Function4/1 -> Trigonometric Function3/2
  Product1/1 -> MATLAB Function3/6(LimitEnable)
  [thetaCorrect] -> Sum16/2, Sum15/2
  MATLAB Function3/1(Eactual) -> Scope18/1, Rate Limiter1/1
  Constant17/1 -> Product1/1
  Sum16/1 -> Trigonometric Function7/1
  Sum13/1 -> Trigonometric Function5/1
  [thetaPcc] -> Scope25/3, Sum8/2
  MATLAB Function2/1(kNext) -> Unit Delay/1
  [deltaActual] -> Scope27/2
  [delta_1] -> Scope25/2, Sum8/1
  [thetaCorrect] -> Sum17/2, Scope26/1
  Sum8/1 -> Scope25/1
  Trigonometric Function1/1 -> Trigonometric Function/2
  [delta_1] -> Scope20/2, Sum18/1
  [Ipcc] -> Scope35/2, Scope19/4
  MATLAB Function/4(scale) -> Scope23/2, Scope19/2
  [delta_1] -> Sum20/1, Sum21/2, Scope21/2
  Sum19/1 -> [thetaCorrect]
  Constant8/1 -> Product/1
  [thetaCorrect] -> MATLAB Function/4(deltaPCC)
  Constant7/1 -> MATLAB Function/6(Imax), Scope16/1
  Product/1 -> MATLAB Function/7(LimitEnable)
  [thetaPcc] -> Scope20/3, Sum18/2
  Delay/1 -> MATLAB Function/5(Imeas)
  [Vpcc] -> Scope17/2, MATLAB Function/3(Vpcc)
  [thetaPcc] -> Sum19/1
  Constant10/1 -> Scope35/3, Scope19/3
  [deltaActual] -> Sum21/1, Scope21/3
  MATLAB Function/2(deltaActual) -> [deltaActual]
  MATLAB Function/3(LimiterActive) -> Scope23/1, [LimiterActive]
  [delta_1] -> Scope22/1
  Constant11/1 -> Sum19/2
  MATLAB Function/1(Eactual) -> Scope17/1, Rate Limiter/1
  [Ecmd] -> Scope17/3, MATLAB Function/1(Ecmd)
  Rate Limiter/1 -> [Eactual]
  Step2/1 -> Product/2
  [thetaCorrect] -> Sum20/2, Scope21/1
  Sum18/1 -> Scope20/1
  [Ipcc] -> Delay/1, Scope16/2
  [delta_1] -> MATLAB Function/2(deltaCmd)
  [deltaActual] -> Scope22/2
  Gain15/1 -> [Vt_V]
  connections:
  Simulink-PS Converter1/RConn1 -- Controlled Voltage Source (Three-Phase)1/LConn1
  Current and Voltage Sensor (Three-Phase)/RConn1 -- PS Selector/LConn1 -- PS-Simulink Converter1/LConn1
  Simulink-PS Converter3/RConn1 -- Controlled Voltage Source (Three-Phase)1/LConn2
  Simulink-PS Converter4/RConn1 -- Circuit Breaker (Three-Phase)/LConn1
  Grounded Neutral (Three-Phase)1/LConn1 -- Circuit Breaker (Three-Phase)/LConn2
  Two-Winding Transformer (Three-Phase)1/RConn1 -- Controlled Voltage Source (Three-Phase)1/RConn1
  Electrical Reference/LConn1 -- Controlled Voltage Source (Three-Phase)/LConn3
  Controlled Voltage Source (Three-Phase)/RConn1 -- Two-Winding Transformer (Three-Phase)/LConn1
  Transmission Line (Three-Phase)/RConn1 -- Two-Winding Transformer (Three-Phase)1/LConn1
  Current and Voltage Sensor (Three-Phase)/LConn1 -- Solver Configuration/RConn1 -- Two-Winding Transformer (Three-Phase)/RConn1
  Current and Voltage Sensor (Three-Phase)/RConn3 -- SPST Switch (Three-Phase)/LConn2 -- Transmission Line (Three-Phase)/LConn1 -- Circuit Breaker (Three-Phase)/RConn1
  Grounded Neutral (Three-Phase)/LConn1 -- RLC (Three-Phase)/LConn1
  Simulink-PS Converter/RConn1 -- Controlled Voltage Source (Three-Phase)/LConn1
  Current and Voltage Sensor (Three-Phase)/RConn2 -- PS-Simulink Converter/LConn1 -- PS Selector1/LConn1
  Simulink-PS Converter2/RConn1 -- Controlled Voltage Source (Three-Phase)/LConn2
  Electrical Reference1/LConn1 -- Controlled Voltage Source (Three-Phase)1/LConn3
  SPST Switch (Three-Phase)/RConn1 -- RLC (Three-Phase)/RConn1
  Simulink-PS Converter5/RConn1 -- SPST Switch (Three-Phase)/LConn1
  "PS Harmonic Estimator (Amplitude, Phase)"/LConn1 -- PS Selector/RConn1
  PS-Simulink Converter2/LConn1 -- "PS Harmonic Estimator (Amplitude, Phase)"/RConn1
  PS-Simulink Converter4/LConn1 -- "PS Harmonic Estimator (Amplitude, Phase)1"/RConn1
  PS-Simulink Converter5/LConn1 -- "PS Harmonic Estimator (Amplitude, Phase)1"/RConn2
  "PS Harmonic Estimator (Amplitude, Phase)1"/LConn1 -- PS Selector1/RConn1
  PS-Simulink Converter3/LConn1 -- "PS Harmonic Estimator (Amplitude, Phase)"/RConn2
